simulink model "hobs_test"  (R2026a)
settings: Solver=VariableStepAuto
settings Model: Creator=dbagn  LastModifiedBy=dbagn

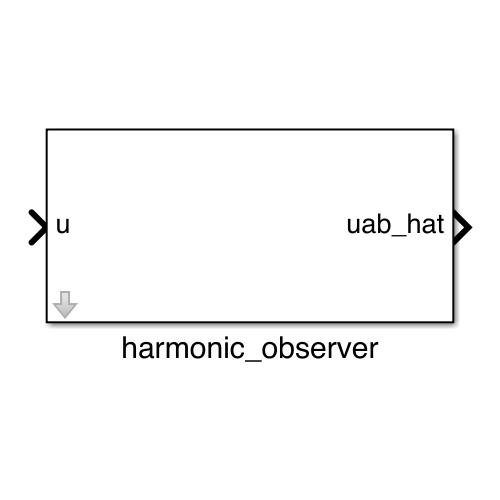
[thumbnail: Simulink's stored preview of the top-level diagram]
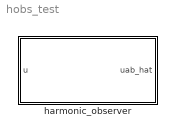
== system hobs_test ==
  harmonic_observer : Subsystem  mask{omega_base=2*pi*50, delta=0.05, pole1=2*pi*50, pole2=2*pi*50*4, ts=250e-6}
      mask init:
      | harmonic_obs = harmonic_observer(omega_base, delta, pole1, pole2, ts);

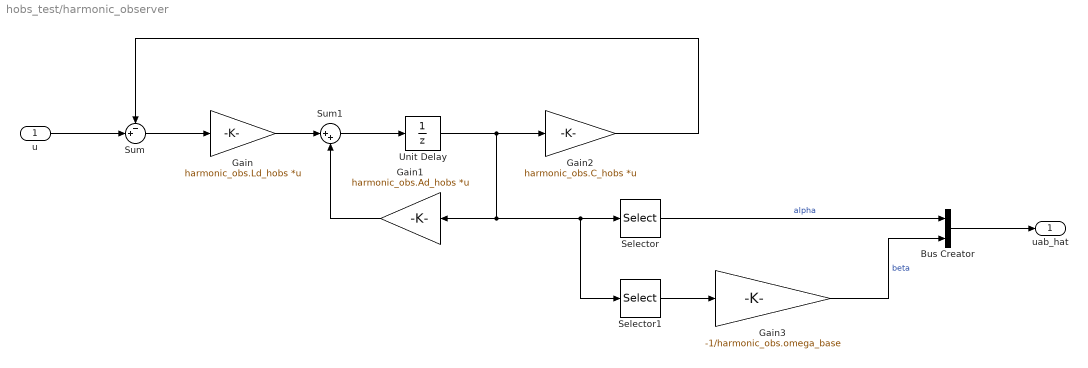
== system hobs_test/harmonic_observer ==
  u : Inport
  Bus Creator : BusCreator  Inputs=2
  Gain : Gain  Gain=harmonic_obs.Ld_hobs  Multiplication=Matrix(K*u)
  Gain1 : Gain  Gain=harmonic_obs.Ad_hobs  Multiplication=Matrix(K*u)
  Gain2 : Gain  Gain=harmonic_obs.C_hobs  Multiplication=Matrix(K*u)
  Gain3 : Gain  Gain=-1/harmonic_obs.omega_base
  Selector : Selector  InputPortWidth=2  IndexOptions=Index vector (dialog)  Indices=1  OutputSizes=1
  Selector1 : Selector  InputPortWidth=2  IndexOptions=Index vector (dialog)  Indices=2  OutputSizes=1
  Sum : Sum  Inputs=-+|
  Sum1 : Sum  Inputs=|++
  Unit Delay : UnitDelay  SampleTime=harmonic_obs.ts
  uab_hat : Outport
  wires:
  u/1 -> Sum/2
  Unit Delay/1 -> Gain2/1, Selector1/1, Selector/1, Gain1/1
  Sum/1 -> Gain/1
  Sum1/1 -> Unit Delay/1
  Gain1/1 -> Sum1/2
  Gain2/1 -> Sum/1
  Selector/1 -> Bus Creator/1  "alpha"
  Gain/1 -> Sum1/1
  Selector1/1 -> Gain3/1
  Gain3/1 -> Bus Creator/2  "beta"
  Bus Creator/1 -> uab_hat/1
